simulink model "sim_model"  (R2023b)
settings: Solver=VariableStepAuto  StartTime=0.0  StopTime=5  RelTol=1e-3
values from neighbouring files (symbols this model uses):
  k = 15    [script.m]
  l_xv = 0.19    [script.m]
  l_yn = 0.31    [script.m]
  l_zv = 0.21    [script.m]
  T = 0.15    [script.m]
settings Model: Creator=user  LastModifiedBy=user

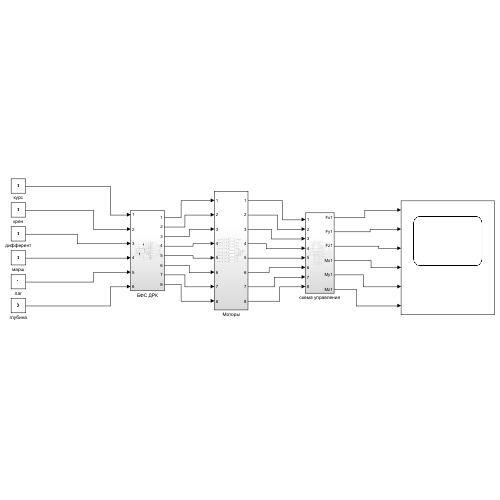
[thumbnail: Simulink's stored preview of the top-level diagram]
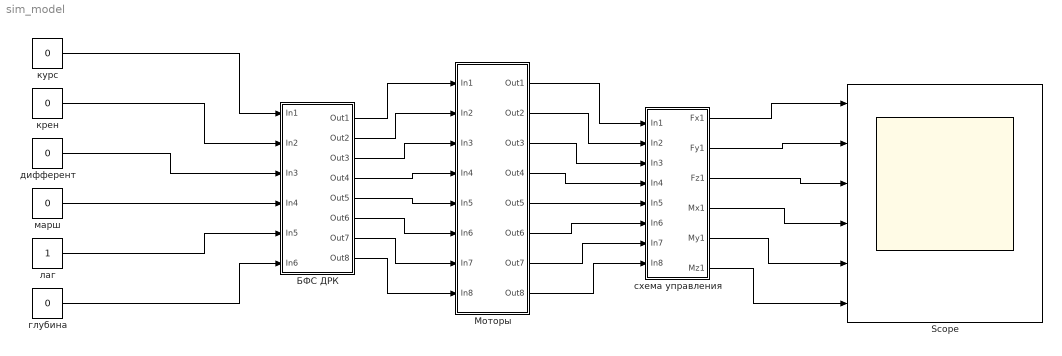
== system sim_model ==
  Scope : Scope  NumInputPorts=6
  БФС ДРК : Subsystem
  Моторы : Subsystem
  глубина : Constant  Value=0
  дифферент : Constant  Value=0
  крен : Constant  Value=0
  курс : Constant  Value=0
  лаг : Constant
  марш : Constant  Value=0
  схема управления : Subsystem
  wires:
  курс/1 -> БФС ДРК/1(In1)
  крен/1 -> БФС ДРК/2(In2)
  дифферент/1 -> БФС ДРК/3(In3)
  марш/1 -> БФС ДРК/4(In4)
  лаг/1 -> БФС ДРК/5(In5)
  глубина/1 -> БФС ДРК/6(In6)
  БФС ДРК/1(Out1) -> Моторы/1(In1)
  БФС ДРК/2(Out2) -> Моторы/2(In2)
  БФС ДРК/3(Out3) -> Моторы/3(In3)
  БФС ДРК/4(Out4) -> Моторы/4(In4)
  БФС ДРК/5(Out5) -> Моторы/5(In5)
  БФС ДРК/6(Out6) -> Моторы/6(In6)
  БФС ДРК/7(Out7) -> Моторы/7(In7)
  БФС ДРК/8(Out8) -> Моторы/8(In8)
  Моторы/1(Out1) -> схема управления/1(In1)
  Моторы/2(Out2) -> схема управления/2(In2)
  Моторы/3(Out3) -> схема управления/3(In3)
  Моторы/4(Out4) -> схема управления/4(In4)
  Моторы/5(Out5) -> схема управления/5(In5)
  Моторы/6(Out6) -> схема управления/6(In6)
  Моторы/7(Out7) -> схема управления/7(In7)
  Моторы/8(Out8) -> схема управления/8(In8)
  схема управления/1(Fx1) -> Scope/1
  схема управления/2(Fy1) -> Scope/2
  схема управления/3(Fz1) -> Scope/3
  схема управления/4(Mx1) -> Scope/4
  схема управления/5(My1) -> Scope/5
  схема управления/6(Mz1) -> Scope/6

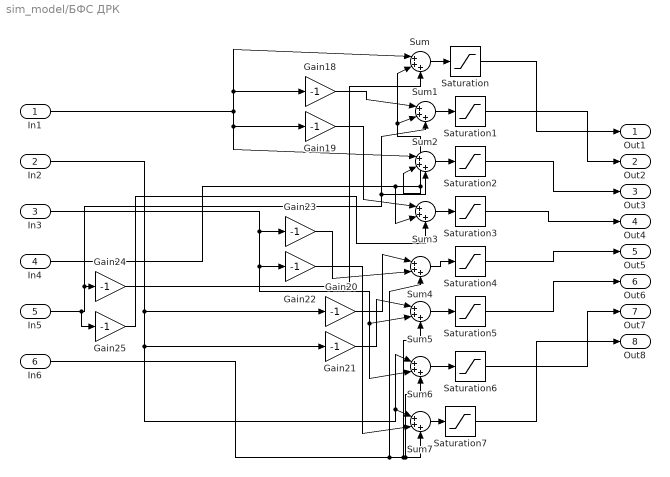
== system sim_model/БФС ДРК ==
  In1 : Inport
  In2 : Inport  Port=2
  In3 : Inport  Port=3
  In4 : Inport  Port=4
  In5 : Inport  Port=5
  In6 : Inport  Port=6
  Gain{18..25} (8 alike) : Gain  Gain=-1
  Saturation{,1..7} (8 alike) : Saturate  UpperLimit=1  LowerLimit=-1
  Sum{,1..7} (8 alike) : Sum  Inputs=|+++
  Out1 : Outport
  Out2 : Outport  Port=2
  Out3 : Outport  Port=3
  Out4 : Outport  Port=4
  Out5 : Outport  Port=5
  Out6 : Outport  Port=6
  Out7 : Outport  Port=7
  Out8 : Outport  Port=8
  wires:
  In3/1 -> Gain23/1, Gain22/1, Sum6/2, Sum5/2
  In4/1 -> Sum1/2, Sum/2, Sum2/2, Sum3/2
  In6/1 -> Sum4/3, Sum5/3, Sum6/3, Sum7/3
  Sum2/1 -> Saturation2/1
  Gain21/1 -> Sum5/1
  Gain20/1 -> Sum4/1
  In1/1 -> Gain18/1, Sum/1, Gain19/1, Sum2/1
  Gain22/1 -> Sum7/2
  Sum6/1 -> Saturation6/1
  Gain24/1 -> Sum/3
  In2/1 -> Gain21/1, Sum6/1, Sum7/1, Gain20/1
  In5/1 -> Gain25/1, Gain24/1, Sum2/3, Sum1/3
  Gain19/1 -> Sum3/1
  Sum4/1 -> Saturation4/1
  Sum/1 -> Saturation/1
  Gain25/1 -> Sum3/3
  Gain18/1 -> Sum1/1
  Sum5/1 -> Saturation5/1
  Gain23/1 -> Sum4/2
  Sum1/1 -> Saturation1/1
  Sum7/1 -> Saturation7/1
  Saturation2/1 -> Out3/1
  Saturation5/1 -> Out6/1
  Sum3/1 -> Saturation3/1
  Saturation3/1 -> Out4/1
  Saturation7/1 -> Out8/1
  Saturation6/1 -> Out7/1
  Saturation/1 -> Out1/1
  Saturation4/1 -> Out5/1
  Saturation1/1 -> Out2/1

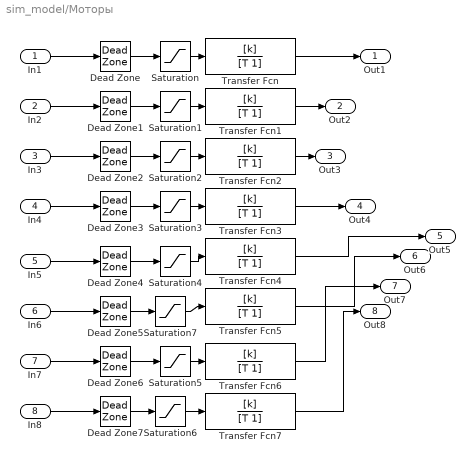
== system sim_model/Моторы ==
  In1 : Inport
  In2 : Inport  Port=2
  In3 : Inport  Port=3
  In4 : Inport  Port=4
  In5 : Inport  Port=5
  In6 : Inport  Port=6
  In7 : Inport  Port=7
  In8 : Inport  Port=8
  Dead Zone{,1..7} (8 alike) : DeadZone
  Saturation{,1..7} (8 alike) : Saturate  UpperLimit=10  LowerLimit=-10
  Transfer Fcn{,1..7} (8 alike) : TransferFcn  Numerator=[k]  Denominator=[T 1]
  Out1 : Outport
  Out2 : Outport  Port=2
  Out3 : Outport  Port=3
  Out4 : Outport  Port=4
  Out5 : Outport  Port=5
  Out6 : Outport  Port=6
  Out7 : Outport  Port=7
  Out8 : Outport  Port=8
  wires:
  Transfer Fcn5/1 -> Out6/1
  Dead Zone4/1 -> Saturation4/1
  Saturation1/1 -> Transfer Fcn1/1
  Transfer Fcn2/1 -> Out3/1
  Saturation/1 -> Transfer Fcn/1
  Dead Zone/1 -> Saturation/1
  Transfer Fcn1/1 -> Out2/1
  Saturation7/1 -> Transfer Fcn5/1
  In5/1 -> Dead Zone4/1
  Saturation4/1 -> Transfer Fcn4/1
  In3/1 -> Dead Zone2/1
  Transfer Fcn3/1 -> Out4/1
  Dead Zone3/1 -> Saturation3/1
  Saturation5/1 -> Transfer Fcn6/1
  In7/1 -> Dead Zone6/1
  Dead Zone6/1 -> Saturation5/1
  Saturation3/1 -> Transfer Fcn3/1
  In8/1 -> Dead Zone7/1
  Saturation2/1 -> Transfer Fcn2/1
  Dead Zone2/1 -> Saturation2/1
  Dead Zone5/1 -> Saturation7/1
  Dead Zone7/1 -> Saturation6/1
  Saturation6/1 -> Transfer Fcn7/1
  Dead Zone1/1 -> Saturation1/1
  Transfer Fcn6/1 -> Out7/1
  Transfer Fcn4/1 -> Out5/1
  In6/1 -> Dead Zone5/1
  In4/1 -> Dead Zone3/1
  Transfer Fcn7/1 -> Out8/1
  In1/1 -> Dead Zone/1
  In2/1 -> Dead Zone1/1
  Transfer Fcn/1 -> Out1/1

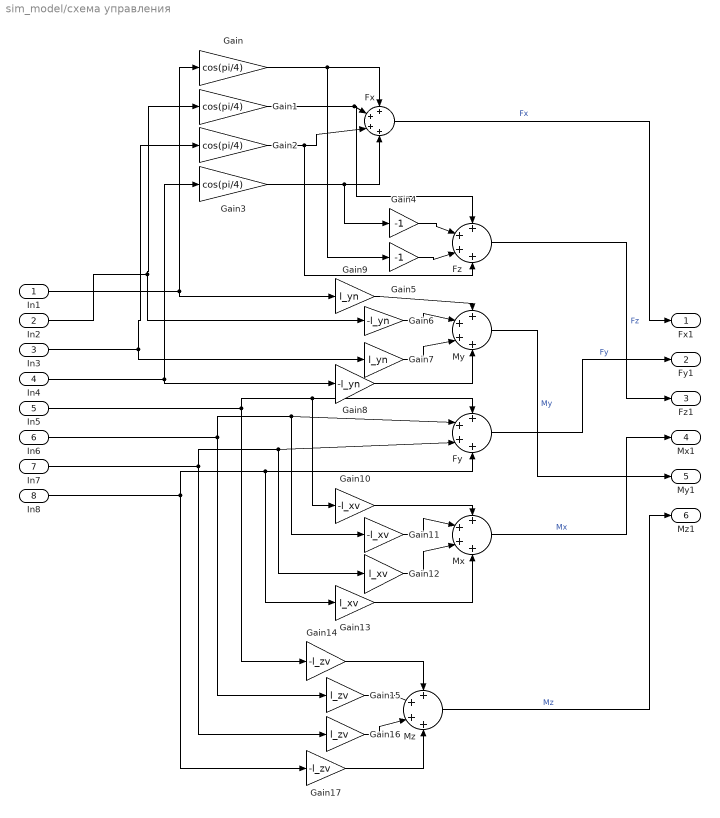
== system sim_model/схема управления ==
  In1 : Inport
  In2 : Inport  Port=2
  In3 : Inport  Port=3
  In4 : Inport  Port=4
  In5 : Inport  Port=5
  In6 : Inport  Port=6
  In7 : Inport  Port=7
  In8 : Inport  Port=8
  Fx : Sum  Inputs=++++
  Fy : Sum  Inputs=++++
  Fz : Sum  Inputs=++++
  Gain{,1..3} (4 alike) : Gain  Gain=cos(pi/4)
  Gain10 : Gain  Gain=-l_xv
  Gain11 : Gain  Gain=-l_xv
  Gain12 : Gain  Gain=l_xv
  Gain13 : Gain  Gain=l_xv
  Gain14 : Gain  Gain=-l_zv
  Gain15 : Gain  Gain=l_zv
  Gain16 : Gain  Gain=l_zv
  Gain17 : Gain  Gain=-l_zv
  Gain4 : Gain  Gain=-1
  Gain5 : Gain  Gain=-1
  Gain6 : Gain  Gain=-l_yn
  Gain7 : Gain  Gain=l_yn
  Gain8 : Gain  Gain=-l_yn
  Gain9 : Gain  Gain=l_yn
  Mx : Sum  Inputs=++++
  My : Sum  Inputs=++++
  Mz : Sum  Inputs=++++
  Fx1 : Outport
  Fy1 : Outport  Port=2
  Fz1 : Outport  Port=3
  Mx1 : Outport  Port=4
  My1 : Outport  Port=5
  Mz1 : Outport  Port=6
  wires:
  Gain1/1 -> Fz/1, Fx/2
  In2/1 -> Gain1/1, Gain6/1
  Gain5/1 -> Fz/3
  In4/1 -> Gain3/1, Gain8/1
  In8/1 -> Gain13/1, Fy/4, Gain17/1
  Gain16/1 -> Mz/3
  In1/1 -> Gain/1, Gain9/1
  Mz/1 -> Mz1/1  "Mz"
  My/1 -> My1/1  "My"
  Gain/1 -> Gain5/1, Fx/1
  In6/1 -> Gain11/1, Fy/2, Gain15/1
  Gain3/1 -> Gain4/1, Fx/4
  Gain4/1 -> Fz/2
  Gain2/1 -> Fz/4, Fx/3
  Gain11/1 -> Mx/2
  In5/1 -> Gain10/1, Fy/1, Gain14/1
  Gain12/1 -> Mx/3
  Gain8/1 -> My/4
  Fz/1 -> Fz1/1  "Fz"
  Gain9/1 -> My/1
  In3/1 -> Gain2/1, Gain7/1
  Gain10/1 -> Mx/1
  Gain17/1 -> Mz/4
  Fx/1 -> Fx1/1  "Fx"
  Gain6/1 -> My/2
  Gain13/1 -> Mx/4
  Gain7/1 -> My/3
  Fy/1 -> Fy1/1  "Fy"
  Gain14/1 -> Mz/1
  Gain15/1 -> Mz/2
  In7/1 -> Gain12/1, Fy/3, Gain16/1
  Mx/1 -> Mx1/1  "Mx"
